simulink subsystem "UHG_UAV_plant_model"  (R2023a)
settings: Solver=VariableStepAuto  StartTime=0.0  StopTime=10.0  RelTol=1e-3
settings Model: Creator=tshintai  LastModifiedBy=tshintai
settings SolverCC: AlgebraicLoopSolver=TrustRegion
settings OptimizationCC: ReuseModelBlockBuffer=off
settings DebuggingCC: UnconnectedInputMsg=warning  UnconnectedOutputMsg=warning  UnconnectedLineMsg=warning
settings ModelReferenceCC: EnableRefExpFcnMdlSchedulingChecks=on
settings RTWCC: DLArmComputeVersion=19.05

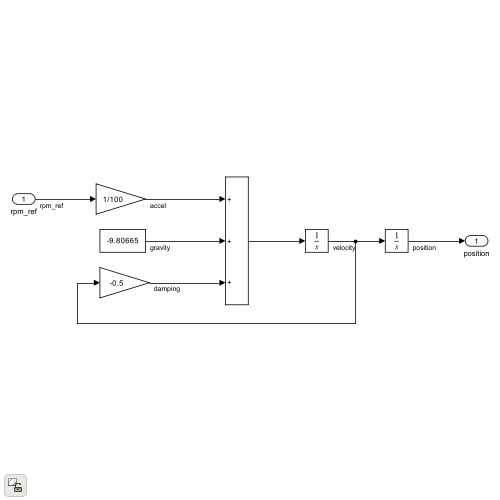
[thumbnail: Simulink's stored preview of the top-level diagram]
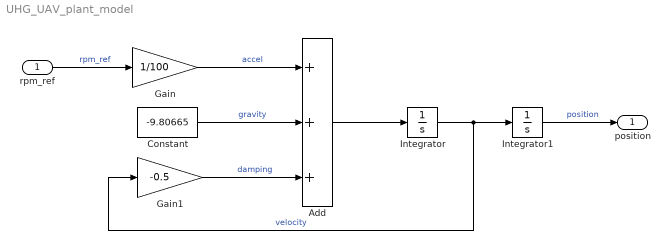
== system UHG_UAV_plant_model ==
  rpm_ref : Inport
  Add : Sum  Inputs=+++
  Constant : Constant  Value=-9.80665
  Gain : Gain  Gain=1/100
  Gain1 : Gain  Gain=-0.5
  Integrator : Integrator
  Integrator1 : Integrator
  position : Outport
  wires:
  rpm_ref/1 -> Gain/1  "rpm_ref"
  Gain/1 -> Add/1  "accel"
  Constant/1 -> Add/2  "gravity"
  Add/1 -> Integrator/1
  Integrator/1 -> Integrator1/1, Gain1/1  "velocity"
  Integrator1/1 -> position/1  "position"
  Gain1/1 -> Add/3  "damping"
